simulink model "modele_palan_obs_sim"  (R2022a)
settings: Solver=FixedStepDiscrete  StartTime=0.0  StopTime=0.3658  FixedStep=Tech  RelTol=1e-3  EnableMultiTasking=on
values from neighbouring files (symbols this model uses):
  data = [0 0 -0.0170399993658 0 -0.00785410404205 0 0.0002 19.9200000763 -0.0170399993658 0.0999961048365 -0.00785410404205 0 ... (10974 elements, 6x1829)]    [p1_obs_1.mat]    (also in p1_obs_2.mat = [0 0 0.0189899988472 0 -0.0329872369766 0 0.0002 19.92000007)
  G = 0.002    [Essai_boucle_ouverte.mat]    (also in PAR_PAL1_IDENT.m; mncarres_incomplet.m; mthgraph.m)
undefined symbols (not defined in the file or in its folder): F, H, Kf, select_file
settings Model: ExtModeArmWhenConnect=off  Creator=ELEPALAN  LastModifiedBy=ELEPALAN
settings SolverCC: AlgebraicLoopSolver=TrustRegion
settings DataIOCC: LimitDataPoints=on  SaveFormat=Array  SignalLoggingSaveFormat=ModelDataLogs  ReturnWorkspaceOutputs=off
settings OptimizationCC: BlockReduction=off  OptimizeBlockIOStorage=off  BufferReuse=off  ExpressionFolding=off  LocalBlockOutputs=off  InitFltsAndDblsToZero=on  LifeSpan=inf
settings DebuggingCC: SaveWithParameterizedLinksMsg=none  UnderspecifiedInitializationDetection=Classic  MergeDetectMultiDrivingBlocksExec=none  SignalResolutionControl=TryResolveAllWithWarning  SolverPrmCheckMsg=warning  MultiTaskDSMMsg=warning  MultiTaskCondExecSysMsg=none  FcnCallInpInsideContextMsg=warning  UnconnectedInputMsg=warning  UnconnectedOutputMsg=warning  UnconnectedLineMsg=warning  SFUnexpectedBacktrackingDiag=warning  SFNoUnconditionalDefaultTransitionDiag=warning  SFExecutionAtInitializationDiag=none  SFMachineParentedDataDiag=warning  ArithmeticOperatorsInVariantConditions=warning
settings HardwareCC: ProdBitPerPointer=32  ProdBitPerSizeT=32  ProdBitPerPtrDiffT=32  ProdLargestAtomicFloat=None  ProdIntDivRoundTo=Undefined  ProdEndianess=Unspecified  ProdWordSize=32  ProdHWDeviceType=32-bit Generic
settings ModelReferenceCC: PropagateSignalLabelsOutOfModel=off
settings RTWCC: Description=xPC Target  SystemTargetFile=xpctarget.tlc  TemplateMakefile=xpc_default_tmf
settings CodeAppCC: StateflowObjectComments=on
settings xpcTargetCC: TargetFcnLib=ansi_tfl_tmw.mat  GenFloatMathFcnCalls=NOT IN USE  TargetLangStandard=C89/C90 (ANSI)  CodeReplacementLibrary=None  MultiwordTypeDef=System defined  DynamicStringBufferSize=256  InferredTypesCompatibility=off  ParMdlRefBuildCompliant=off  CompOptLevelCompliant=off  ConcurrentExecutionCompliant=off  CombineSignalStateStructs=off  GroupInternalDataByFunction=off  CodeInterfacePackaging=Nonreusable function  RemoveDisableFunc=off  RemoveResetFunc=off  CastingMode=Nominal  MATLABClassNameForMDSCustomization=Simulink.SoftwareTarget.TargetSpecificTriggerConfigurationBase  MDXCompliant=off  GRTInterface=on  GenerateAllocFcn=off  UseToolchainInfoCompliant=off  GenerateSharedConstants=on  CoderGroups=[]  AccessMethods=[]  LookupTableObjectStructAxisOrder=1,2,3,4,...  LUTObjectStructOrderExplicitValues=Size,Breakpoints,Table  LUTObjectStructOrderEvenSpacing=Size,Breakpoints,Table  ArrayLayout=Column-major  UnsupportedSFcnMsg=error  ERTHeaderFileRootName=$R$E  ERTSourceFileRootName=$R$E  ERTDataFileRootName=$R_data  OptimizeReductions=off  RL32LogBufSizeModifier=1000000
settings ConfigComp: CovMetricSettings=dw  CovSaveCumulativeToWorkspaceVar=on  CovSaveSingleToWorkspaceVar=on

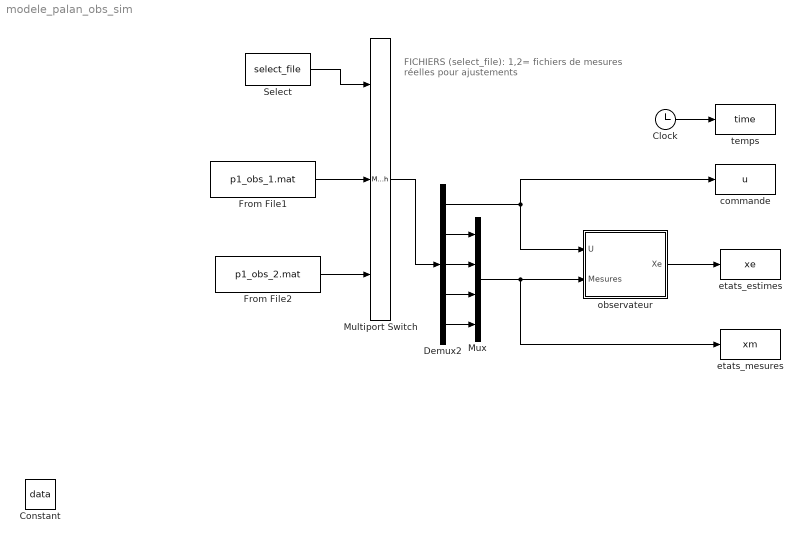
== system modele_palan_obs_sim ==
  note: FICHIERS (select_file):
      | 1,2= fichiers de mesures réelles pour ajustements
  Clock : Clock
  Constant : Constant  Value=data
  Demux2 : Demux  Outputs=5
  From File1 : FromFile  FileName=p1_obs_1.mat
  From File2 : FromFile  FileName=p1_obs_2.mat
  Multiport Switch : MultiPortSwitch  Inputs=2  OutDataTypeStr=Inherit: Same as first data input  SaturateOnIntegerOverflow=off  InputSameDT=off
  Mux : Mux
  Select : Constant  Value=select_file
  commande : ToWorkspace  VariableName=u  SampleTime=-1
  etats_estimes : ToWorkspace  VariableName=xe  SampleTime=-1
  etats_mesures : ToWorkspace  VariableName=xm  SampleTime=-1
  observateur : Subsystem
  temps : ToWorkspace  VariableName=time  SampleTime=-1
  wires:
  Mux/1 -> observateur/2(Mesures), etats_mesures/1
  observateur/1(Xe) -> etats_estimes/1
  Clock/1 -> temps/1
  Demux2/2 -> Mux/1
  Demux2/3 -> Mux/2
  Demux2/4 -> Mux/3
  Demux2/5 -> Mux/4
  Demux2/1 -> commande/1, observateur/1(U)
  From File2/1 -> Multiport Switch/3
  From File1/1 -> Multiport Switch/2
  Select/1 -> Multiport Switch/1
  Multiport Switch/1 -> Demux2/1

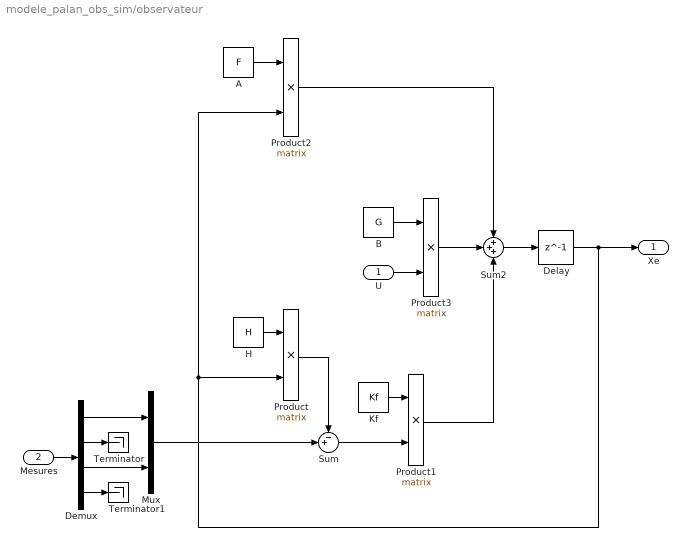
== system modele_palan_obs_sim/observateur ==
  U : Inport
  Mesures : Inport  Port=2
  A : Constant  Value=F  SampleTime=-1
  B : Constant  Value=G  SampleTime=-1
  Delay : Delay  DelayLength=1
  Demux : Demux
  H : Constant  Value=H
  Kf : Constant  Value=Kf
  Mux : Mux  Inputs=2
  Product{,1..3} (4 alike) : Product  Multiplication=Matrix(*)  RndMeth=Zero
  Sum : Sum  Inputs=-+|
  Sum2 : Sum  Inputs=+++
  Terminator : Terminator
  Terminator1 : Terminator
  Xe : Outport
  wires:
  H/1 -> Product/1
  Product/1 -> Sum/1
  Sum/1 -> Product1/2
  U/1 -> Product3/2
  Product3/1 -> Sum2/2
  Product2/1 -> Sum2/1
  Product1/1 -> Sum2/3
  Sum2/1 -> Delay/1
  Delay/1 -> Xe/1, Product/2, Product2/2
  A/1 -> Product2/1
  B/1 -> Product3/1
  Kf/1 -> Product1/1
  Mesures/1 -> Demux/1
  Demux/3 -> Mux/2
  Demux/1 -> Mux/1
  Mux/1 -> Sum/2
  Demux/2 -> Terminator/1
  Demux/4 -> Terminator1/1
